simulink model "Closed_loop_buck_boost_test"  (R2024b)
settings: Solver=VariableStepAuto  StartTime=0.0  StopTime=10.0  RelTol=1e-3
libraries: spsSeriesRLCBranchLib x4, spsCurrentMeasurementLib x2, spsDiodeLib x2, simulink x2, spsMosfetLib x2, spsVoltageMeasurementLib x2, spsControlledVoltageSourceLib x1, spsGroundLib x1, slpidlib x1, spspowerguiLib x1
settings Model: VariantFading=off  Creator=Abdal  LastModifiedBy=Abdal
settings DebuggingCC: AlgebraicLoopMsg=none

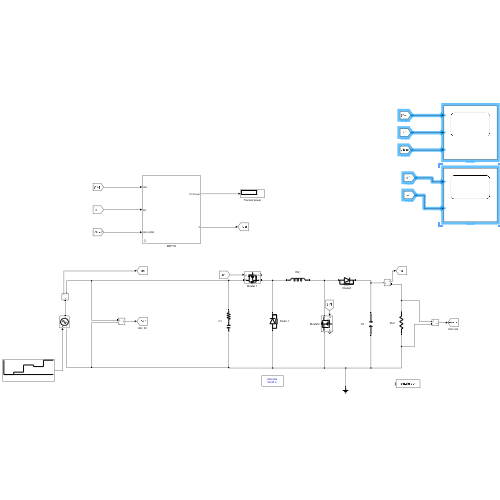
[thumbnail: Simulink's stored preview of the top-level diagram]
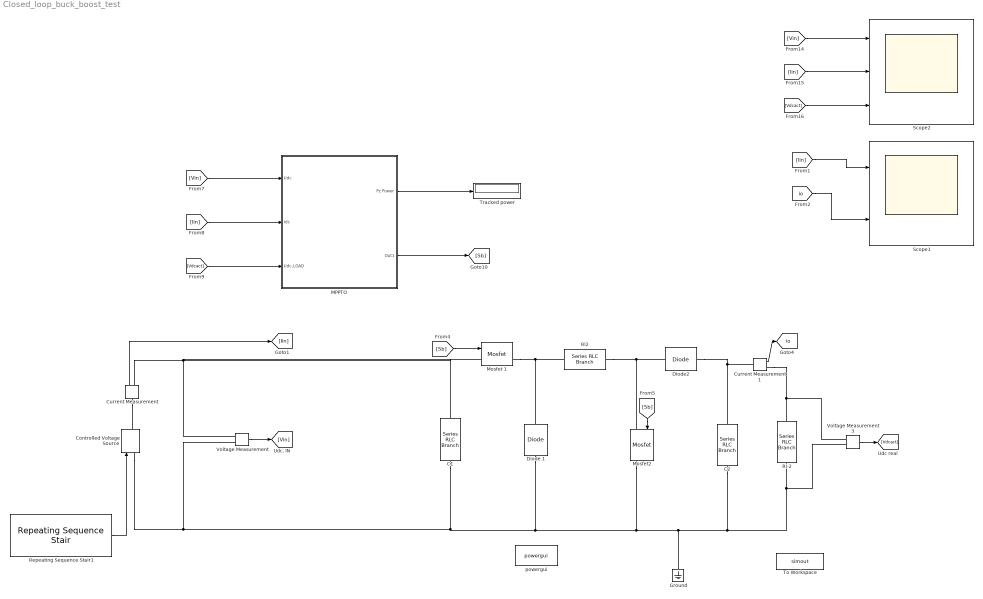
== system Closed_loop_buck_boost_test ==
  C1 : spsSeriesRLCBranchLib/Series RLC Branch  LConnTagsString=__new0  RConnTagsString=__new0  BranchType=RC  Resistance=70  Inductance=1e-3  SetiL0=off  InitialCurrent=0  Capacitance=120  Setx0=off  InitialVoltage=0  Measurements=None
  C2 : spsSeriesRLCBranchLib/Series RLC Branch  LConnTagsString=__new0  RConnTagsString=__new0  BranchType=C  Resistance=1  Inductance=1e-3  SetiL0=off  InitialCurrent=0  Capacitance=200  Setx0=off  InitialVoltage=0  Measurements=None
  Controlled Voltage Source : spsControlledVoltageSourceLib/Controlled Voltage Source  Initialize=on  Source_Type=DC  Amplitude=0  Phase=0  Frequency=0  Measurements=Voltage
  Current Measurement : spsCurrentMeasurementLib/Current Measurement  PhasorSimulation=off  OutputType=Complex  PSBequivalent=0
  Current Measurement1 : spsCurrentMeasurementLib/Current Measurement  PhasorSimulation=off  OutputType=Complex  PSBequivalent=0
  "Diode 1 " : spsDiodeLib/Diode  Ron=0.001  Lon=0  Vf=0.8  IC=0  UseSnubber=0  Rs=500  Cs=250e-9  Measurements=off
  Diode2 : spsDiodeLib/Diode  Ron=0.001  Lon=0  Vf=0.8  IC=0  UseSnubber=0  Rs=500  Cs=250e-9  Measurements=off
  Ground : spsGroundLib/Ground  LConnTagsString=a
  MPPTO : Subsystem  mask{Dstep=0.01}
      mask prompts: Dstep "Perturbation step ΔD"
  "Mosfet 1 " : spsMosfetLib/Mosfet  Ron=0.1  Lon=0  Rd=0.01  Vfd=0  IC=0  Rs=1e5  Cs=inf  Measurements=on
  Mosfet2 : spsMosfetLib/Mosfet  Ron=0.1  Lon=0  Rd=0.01  Vfd=0  IC=0  Rs=1e5  Cs=inf  Measurements=on
  Repeating Sequence Stair1 : simulink/Sources/Repeating Sequence Stair  OutValues=[0 10 40 34 60]  tsamp=2  OutMin=[]  OutMax=[]  OutDataTypeStr=double  OutputDataTypeScalingMode=double  OutDataType=fixdt(0,8)  ConRadixGroup=Best Precision: Vector-wise  OutScaling=2^-12
  Rl-2 : spsSeriesRLCBranchLib/Series RLC Branch  LConnTagsString=__new0  RConnTagsString=__new0  BranchType=R  Resistance=40  Inductance=1e-3  SetiL0=off  InitialCurrent=0  Capacitance=1e-6  Setx0=off  InitialVoltage=0  Measurements=None
  Rl2 : spsSeriesRLCBranchLib/Series RLC Branch  LConnTagsString=__new0  RConnTagsString=__new0  BranchType=L  Resistance=1  Inductance=350  SetiL0=on  InitialCurrent=6  Capacitance=1e-6  Setx0=off  InitialVoltage=0  Measurements=None
  Scope1 : Scope  NumInputPorts=2
  Scope2 : Scope  NumInputPorts=3
  To Workspace : ToWorkspace  VariableName=simout  SaveFormat=Structure With Time  SampleTime=-1
  Tracked power : Display
  Voltage Measurement : spsVoltageMeasurementLib/Voltage Measurement  PhasorSimulation=off  OutputType=Complex  PSBequivalent=0
  Voltage Measurement3 : spsVoltageMeasurementLib/Voltage Measurement  PhasorSimulation=off  OutputType=Complex  PSBequivalent=0
  powergui : spspowerguiLib/powergui  Priority=1  SimulationMode=Discrete  SampleTime=50e-6  frequency=60  Iterations=50  frequencyindice=0  Pbase=100e6  ErrMax=1e-4  UnitsV=kV  UnitsW=MW  buscounter=0  FunctionMessages=off  echomessages=off  EnableUseOfTLC=off  CurrentSourceSwitches=off  DisableSnubberDevices=off  DisableRonSwitches=off  DisableVfSwitches=off  DisplayEquations=off  AutomaticDiscreteSolvers=off  SolverType=Tustin/Backward Euler (TBE)  Interpol=off  ExternalGateDelay=off  methode=off  Ts=100  x0status=blocks  SPID=on  SwTol=0  HookPort=off  NonlinearTolerance=1e-4  nMaxIteration=100  ContinueOnMaxIteration=off  RestoreLinks=warning  ResistiveCurrentMeasurement=off  Frange=[0:2:500]  Ylog=off  Xlog=on  ShowGrid=off  save=off  variable=ZData  structure=0  ZoomFFT=off  StartTime=0.0  cycles=1  DisplayStyle=1  fundamental=60  FreqAxis=off  MaxFrequency=1000  frequencyindicesteady=1  RmsSteady=1  display=off
  tag scope: io=global
  wires:
  [Sb] -> "Mosfet 1 "/1
  [Sb] -> Mosfet2/1
  Current Measurement1/1 -> [io]
  Voltage Measurement3/1 -> [Vdcact]
  [Vin] -> Scope2/1
  [Iin] -> Scope2/2
  [Vdcact] -> Scope2/3
  Voltage Measurement/1 -> [Vin]
  Current Measurement/1 -> [Iin]
  MPPTO/2(Out1) -> [Sb]
  [Vdcact] -> MPPTO/3(Udc,LOAD)
  [Iin] -> MPPTO/2(Idc)
  MPPTO/1(Pz Power) -> Tracked power/1
  [Vin] -> MPPTO/1(Udc)
  Repeating Sequence Stair1/1 -> Controlled Voltage Source/1
  [Iin] -> Scope1/1
  [io] -> Scope1/2
  connections:
  Controlled Voltage Source/LConn1 -- Ground/LConn1 -- C2/RConn1 -- Voltage Measurement3/LConn2 -- Rl-2/RConn1 -- Mosfet2/RConn1 -- "Diode 1 "/LConn1 -- C1/RConn1 -- Voltage Measurement/LConn2
  "Diode 1 "/RConn1 -- Rl2/RConn1 -- "Mosfet 1 "/RConn1
  Rl2/LConn1 -- Diode2/LConn1 -- Mosfet2/LConn1
  Diode2/RConn1 -- Current Measurement1/LConn1 -- C2/LConn1
  Current Measurement1/RConn1 -- Voltage Measurement3/LConn1 -- Rl-2/LConn1
  Voltage Measurement/LConn1 -- "Mosfet 1 "/LConn1 -- C1/LConn1 -- Current Measurement/RConn1
  Current Measurement/LConn1 -- Controlled Voltage Source/RConn1

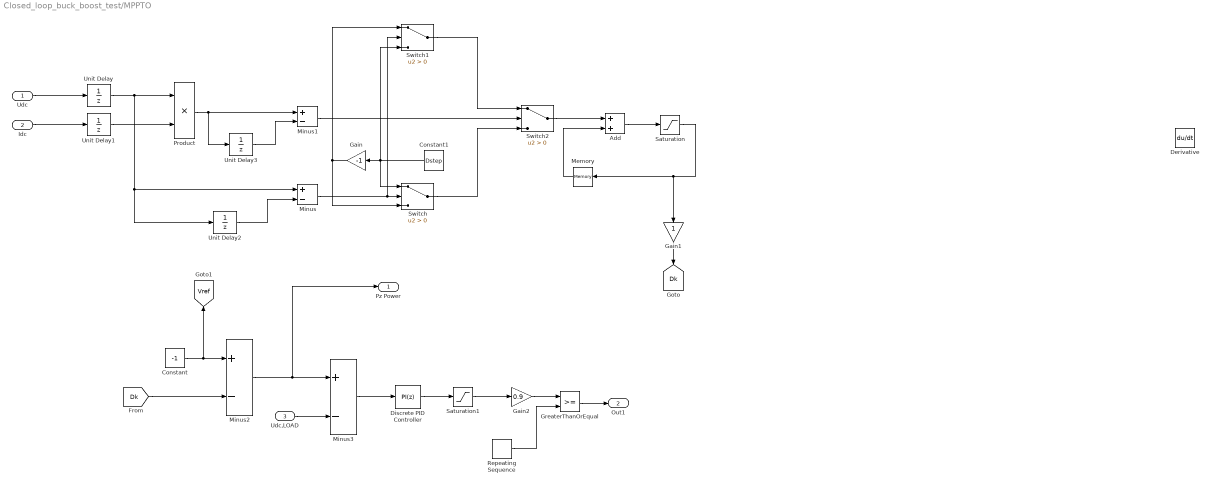
== system Closed_loop_buck_boost_test/MPPTO ==
  Udc : Inport
  Idc : Inport  Port=2
  Udc,LOAD : Inport  Port=3
  Add : Sum
  Constant : Constant  Value=-1  VectorParams1D=off
  Constant1 : Constant  Value=Dstep
  Derivative : Derivative
  Discrete PID Controller : slpidlib/PID Controller  Controller=PI  Form=Ideal  TimeDomain=Discrete-time  UseExternalTs=off  SampleTime=-1  IntegratorMethod=Forward Euler  FilterMethod=Forward Euler  ControllerParametersSource=internal  P=0.0143  I=0.0357  UseKiTs=off  D=0  UseExternalDerivativeSource=off  N=100  UseFilter=on  TunerSelectOption=Frequency Response Based  InitialConditionSource=internal  InitialConditionForIntegrator=0  InitialConditionForFilter=0  DifferentiatorICPrevScaledInput=0  ExternalReset=none  TrackingMode=off  Kt=1  LimitOutput=off  SatLimitsSource=internal  UpperSaturationLimit=inf  LowerSaturationLimit=-inf  LinearizeAsGain=off  AntiWindupMode=none  Kb=1  LimitIntegrator=off  UpperIntegratorSaturationLimit=inf  LowerIntegratorSaturationLimit=-inf  POutMin=[]  POutMax=[]  IOutMin=[]  IOutMax=[]  DOutMin=[]  DOutMax=[]  NOutMin=[]  NOutMax=[]  SumOutMin=[]  SumOutMax=[]  SaturationOutMin=[]  SaturationOutMax=[]  PParamMin=[]  PParamMax=[]  IParamMin=[]  IParamMax=[]  DParamMin=[]  DParamMax=[]  NParamMin=[]  NParamMax=[]  KbParamMin=[]  KbParamMax=[]  KtParamMin=[]  KtParamMax=[]  KbOutMin=[]  KbOutMax=[]  KtOutMin=[]  KtOutMax=[]  IntegratorOutMin=[]  IntegratorOutMax=[]  FilterOutMin=[]  FilterOutMax=[]  SumI1OutMin=[]  SumI1OutMax=[]  SumI2OutMin=[]  SumI2OutMax=[]  SumI3OutMin=[]  SumI3OutMax=[]  SumI4OutMin=[]  SumI4OutMax=[]  SumDOutMin=[]  SumDOutMax=[]  DifferentiatorOutMin=[]  DifferentiatorOutMax=[]  FilterDiffOutCoefMin=[]  FilterDiffOutCoefMax=[]  ReciprocalOutMin=[]  ReciprocalOutMax=[]  SumDenOutMin=[]  SumDenOutMax=[]  SumNumOutMin=[]  SumNumOutMax=[]  DivideOutMin=[]  DivideOutMax=[]  UdiffTsProdOutMin=[]  UdiffTsProdOutMax=[]  NTsProdOutMin=[]  NTsProdOutMax=[]  UintegralTsProdOutMin=[]  UintegralTsProdOutMax=[]  UngainTsProdOutMin=[]  UngainTsProdOutMax=[]  ClampingZeroOutDataTypeStr=Inherit: Inherit via back propagation  ClampingZeroOutMin=[]  ClampingZeroOutMax=[]  FilterDenConstantOutDataTypeStr=Inherit: Inherit via back propagation  FilterDenConstantOutMin=[]  FilterDenConstantOutMax=[]  PCopyOutDataTypeStr=Inherit: Inherit via back propagation  PCopyOutMin=[]  PCopyOutMax=[]  NCopyOutDataTypeStr=Inherit: Inherit via back propagation  NCopyOutMin=[]  NCopyOutMax=[]  IntegratorContinuousStateAttributes=''  IntegratorStateMustResolveToSignalObject=off  IntegratorRTWStateStorageClass=Auto  FilterContinuousStateAttributes=''  FilterStateMustResolveToSignalObject=off  FilterRTWStateStorageClass=Auto  ParallelPVariant=Passthrough  IdealPVariant=InternalParameters  IVariant=InternalParameters  DVariant=Disabled  IntegratorVariant=Discrete  SatVariant=Disabled  AWVariant=Passthrough  PCopyVariant=Disabled  TRVariant=Disabled  FdbkBlocksVariant=Forward  IdealPFdbkVariant=Disabled  SatFdbkVariant=Disabled  DerivativeFilterVariant=Disabled  NVariant=Disabled  NCopyVariant=Disabled_SignalSpec  FilterICVariant=Disabled  IntegratorICVariant=InternalICs  ExternalResetVariant=Disabled  TRSumVariant=Passthrough  SumFdbkVariant=Disabled  SumVariant=Sum_PI  TsampFilterVariant=InternalTs  TsampNgainVariant=Passthrough  TsampIntegralVariant=Disabled_SignalSpec  ExternalSaturationOutDataTypeStr=Inherit: Same as second input  DerivativeSourceVariant=Disabled  PreIntVariant=InternalPreInt
  Gain : Gain  Gain=-1
  Gain1 : Gain
  Gain2 : Gain  Gain=0.9
  GreaterThanOrEqual : RelationalOperator  OutDataTypeStr=boolean  RndMeth=Simplest  InputSameDT=off
  Memory : Memory
  Minus{,1..3} (4 alike) : Sum  Inputs=+-
  Product : Product
  Repeating Sequence : simulink/Sources/Repeating Sequence  rep_seq_t=[0 2]  rep_seq_y=[0 2]
  Saturation : Saturate  UpperLimit=0.6  LowerLimit=0.4
  Saturation1 : Saturate  UpperLimit=0.6  LowerLimit=0.4
  Switch : Switch  Criteria=u2 > Threshold  SaturateOnIntegerOverflow=off  InputSameDT=off
  Switch1 : Switch  Criteria=u2 > Threshold  SaturateOnIntegerOverflow=off  InputSameDT=off
  Switch2 : Switch  Criteria=u2 > Threshold  SaturateOnIntegerOverflow=off  InputSameDT=off
  Unit Delay{,1..3} (4 alike) : UnitDelay  SampleTime=-1  HasFrameUpgradeWarning=on
  Pz Power : Outport
  Out1 : Outport  Port=2
  tag scope: Dk=global, Vref=global
  wires:
  Udc/1 -> Unit Delay/1
  Idc/1 -> Unit Delay1/1
  Unit Delay/1 -> Product/1, Minus/1, Unit Delay2/1
  Unit Delay1/1 -> Product/2
  Unit Delay2/1 -> Minus/2
  Minus/1 -> Switch1/2, Switch/2
  Unit Delay3/1 -> Minus1/2
  Minus1/1 -> Switch2/2
  Switch1/1 -> Switch2/1
  Switch/1 -> Switch2/3
  Switch2/1 -> Add/1
  Add/1 -> Saturation/1
  Gain/1 -> Switch/3, Switch1/1
  Saturation/1 -> Gain1/1, Memory/1
  Memory/1 -> Add/2
  Constant1/1 -> Switch/1, Switch1/3, Gain/1
  Gain1/1 -> [Dk]
  Product/1 -> Unit Delay3/1, Minus1/1
  [Dk] -> Minus2/2
  Constant/1 -> Minus2/1, [Vref]
  Minus2/1 -> Pz Power/1, Minus3/1
  Udc,LOAD/1 -> Minus3/2
  Minus3/1 -> Discrete PID Controller/1
  Discrete PID Controller/1 -> Saturation1/1
  Saturation1/1 -> Gain2/1
  Gain2/1 -> GreaterThanOrEqual/1
  Repeating Sequence/1 -> GreaterThanOrEqual/2
  GreaterThanOrEqual/1 -> Out1/1
